simulink model "ModelLLCController"  (R2026a)
settings: Solver=ode23t  StopTime=5e-3  FixedStep=1e-4  MaxStep=1/(10*llcCompensator.resonantFrequency)  AbsTol=1e-3
PreLoadFcn:
  | % Parameterize the model
  | 
  | if ~exist('LLCDesign', 'var')
  | LLCConverterDefaultInputParameters;
  | end
undefined symbols (not defined in the file or in its folder): llcCompensator, LLCController
libraries: fl_lib x52, nesl_utility x34, ee_lib x27, ConverterLibrary x1
(part 3 of 4)

== system ModelLLCController/LLC Converter Power Circuit/LLC Primary Inverter and Resonant Tank/LLC Simplified Model/Inverter/Half Bridge Converter ==
  G1 : Inport
  G2 : Inport  Port=2
  Diode1 : fl_lib/Electrical/Electrical Elements/Diode  Vf=VfBody V  Ron=RdBody Ohm  Goff=GdBody 1/Ohm  i_specify=off  i_priority=None  i=0 A  i_nominal_specify=off  i_nominal_value=1  i_nominal_unit=A  v_specify=off  v_priority=None  v=0 V  v_nominal_specify=off  v_nominal_value=1  v_nominal_unit=V
  Diode2 : fl_lib/Electrical/Electrical Elements/Diode  Vf=VfBody V  Ron=RdBody Ohm  Goff=GdBody 1/Ohm  i_specify=off  i_priority=None  i=0 A  i_nominal_specify=off  i_nominal_value=1  i_nominal_unit=A  v_specify=off  v_priority=None  v=0 V  v_nominal_specify=off  v_nominal_value=1  v_nominal_unit=V
  Simulink-PS Converter1 : nesl_utility/Simulink-PS Converter  PhysicalDomain=network_engine_domain  SubClassName=ps_input  LeftPortType=input  RightPortType=output  PseudoPeriodic=off  Frequencies=[]  NoiseDistribution=none  NoiseParameters=[]  Unit=1  AffineConversion=off  FilteringAndDerivatives=provide  SimscapeFilterOrder=1  InputFilterTimeConstant=0.001  UdotUserProvided=0
  Simulink-PS Converter2 : nesl_utility/Simulink-PS Converter  PhysicalDomain=network_engine_domain  SubClassName=ps_input  LeftPortType=input  RightPortType=output  PseudoPeriodic=off  Frequencies=[]  NoiseDistribution=none  NoiseParameters=[]  Unit=1  AffineConversion=off  FilteringAndDerivatives=provide  SimscapeFilterOrder=1  InputFilterTimeConstant=0.001  UdotUserProvided=0
  Switch : fl_lib/Electrical/Electrical Elements/Switch  R_closed=RdsOn Ohm  G_open=GdsOff 1/Ohm  Threshold=Vth  i_specify=off  i_priority=None  i=0 A  i_nominal_specify=off  i_nominal_value=1  i_nominal_unit=A  v_specify=off  v_priority=None  v=0 V  v_nominal_specify=off  v_nominal_value=1  v_nominal_unit=V
  Switch1 : fl_lib/Electrical/Electrical Elements/Switch  R_closed=RdsOn Ohm  G_open=GdsOff 1/Ohm  Threshold=Vth  i_specify=off  i_priority=None  i=0 A  i_nominal_specify=off  i_nominal_value=1  i_nominal_unit=A  v_specify=off  v_priority=None  v=0 V  v_nominal_specify=off  v_nominal_value=1  v_nominal_unit=V
  P1 : PMIOPort  Side=Left
  N1 : PMIOPort  Port=2  Side=Left
  P2 : PMIOPort  Port=3  Side=Right
  N2 : PMIOPort  Port=4  Side=Right
  wires:
  G1/1 -> Simulink-PS Converter1/1
  G2/1 -> Simulink-PS Converter2/1
  connections:
  Switch/RConn2 -- Diode2/RConn1 -- P1/RConn1
  Diode2/LConn1 -- Switch/LConn1 -- P2/RConn1 -- Switch1/RConn2 -- Diode1/RConn1
  N1/RConn1 -- Switch1/LConn1 -- Diode1/LConn1 -- N2/RConn1
  Switch1/RConn1 -- Simulink-PS Converter2/RConn1
  Simulink-PS Converter1/RConn1 -- Switch/RConn1

== system ModelLLCController/LLC Converter Power Circuit/LLC Primary Inverter and Resonant Tank/LLC Simplified Model/Inverter/Iin ==
  Current Sensor : fl_lib/Electrical/Electrical Sensors/Current Sensor
  PS-Simulink Converter : nesl_utility/PS-Simulink Converter  PhysicalDomain=network_engine_domain  SubClassName=ps_output  LeftPortType=input  RightPortType=output  PseudoPeriodic=off  Frequencies=[]  VectorFormat=inherit  Unit=inherit  AffineConversion=off
  + : PMIOPort  Side=Left
  - : PMIOPort  Port=2  Side=Right
  I : Outport
  wires:
  PS-Simulink Converter/1 -> I/1
  connections:
  Current Sensor/RConn2 -- -/RConn1
  +/RConn1 -- Current Sensor/LConn1
  Current Sensor/RConn1 -- PS-Simulink Converter/LConn1

== system ModelLLCController/LLC Converter Power Circuit/LLC Primary Inverter and Resonant Tank/LLC Simplified Model/Inverter/Vin ==
  PS-Simulink Converter : nesl_utility/PS-Simulink Converter  PhysicalDomain=network_engine_domain  SubClassName=ps_output  LeftPortType=input  RightPortType=output  PseudoPeriodic=off  Frequencies=[]  VectorFormat=inherit  Unit=inherit  AffineConversion=off
  Voltage Sensor : fl_lib/Electrical/Electrical Sensors/Voltage Sensor
  + : PMIOPort  Side=Left
  - : PMIOPort  Port=2  Side=Right
  V : Outport
  wires:
  PS-Simulink Converter/1 -> V/1
  connections:
  Voltage Sensor/RConn2 -- -/RConn1
  Voltage Sensor/LConn1 -- +/RConn1
  PS-Simulink Converter/LConn1 -- Voltage Sensor/RConn1

== system ModelLLCController/LLC Converter Power Circuit/LLC Primary Inverter and Resonant Tank/LLC Simplified Model/Resonant Tank/Ip ==
  Current Sensor : fl_lib/Electrical/Electrical Sensors/Current Sensor
  PS-Simulink Converter : nesl_utility/PS-Simulink Converter  PhysicalDomain=network_engine_domain  SubClassName=ps_output  LeftPortType=input  RightPortType=output  PseudoPeriodic=off  Frequencies=[]  VectorFormat=inherit  Unit=inherit  AffineConversion=off
  + : PMIOPort  Side=Left
  - : PMIOPort  Port=2  Side=Right
  I : Outport
  wires:
  PS-Simulink Converter/1 -> I/1
  connections:
  Current Sensor/RConn2 -- -/RConn1
  +/RConn1 -- Current Sensor/LConn1
  Current Sensor/RConn1 -- PS-Simulink Converter/LConn1

== system ModelLLCController/LLC Converter Power Circuit/LLC Primary Inverter and Resonant Tank/LLC Simplified Model/Resonant Tank/Is ==
  Current Sensor : fl_lib/Electrical/Electrical Sensors/Current Sensor
  PS-Simulink Converter : nesl_utility/PS-Simulink Converter  PhysicalDomain=network_engine_domain  SubClassName=ps_output  LeftPortType=input  RightPortType=output  PseudoPeriodic=off  Frequencies=[]  VectorFormat=inherit  Unit=inherit  AffineConversion=off
  + : PMIOPort  Side=Left
  - : PMIOPort  Port=2  Side=Right
  I : Outport
  wires:
  PS-Simulink Converter/1 -> I/1
  connections:
  Current Sensor/RConn2 -- -/RConn1
  +/RConn1 -- Current Sensor/LConn1
  Current Sensor/RConn1 -- PS-Simulink Converter/LConn1

== system ModelLLCController/LLC Converter Power Circuit/LLC Primary Inverter and Resonant Tank/LLC Simplified Model/Resonant Tank/Vp ==
  PS-Simulink Converter : nesl_utility/PS-Simulink Converter  PhysicalDomain=network_engine_domain  SubClassName=ps_output  LeftPortType=input  RightPortType=output  PseudoPeriodic=off  Frequencies=[]  VectorFormat=inherit  Unit=inherit  AffineConversion=off
  Voltage Sensor : fl_lib/Electrical/Electrical Sensors/Voltage Sensor
  + : PMIOPort  Side=Left
  - : PMIOPort  Port=2  Side=Right
  V : Outport
  wires:
  PS-Simulink Converter/1 -> V/1
  connections:
  Voltage Sensor/RConn2 -- -/RConn1
  Voltage Sensor/LConn1 -- +/RConn1
  PS-Simulink Converter/LConn1 -- Voltage Sensor/RConn1

== system ModelLLCController/LLC Converter Power Circuit/LLC Primary Inverter and Resonant Tank/LLC Simplified Model/Resonant Tank/Vs ==
  PS-Simulink Converter : nesl_utility/PS-Simulink Converter  PhysicalDomain=network_engine_domain  SubClassName=ps_output  LeftPortType=input  RightPortType=output  PseudoPeriodic=off  Frequencies=[]  VectorFormat=inherit  Unit=inherit  AffineConversion=off
  Voltage Sensor : fl_lib/Electrical/Electrical Sensors/Voltage Sensor
  + : PMIOPort  Side=Left
  - : PMIOPort  Port=2  Side=Right
  V : Outport
  wires:
  PS-Simulink Converter/1 -> V/1
  connections:
  Voltage Sensor/RConn2 -- -/RConn1
  Voltage Sensor/LConn1 -- +/RConn1
  PS-Simulink Converter/LConn1 -- Voltage Sensor/RConn1

== system ModelLLCController/LLC Converter Power Circuit/Rectifier/Rectifier Bridge/Centre-Tap Ideal Diode/Is ==
  Current Sensor : fl_lib/Electrical/Electrical Sensors/Current Sensor
  PS-Simulink Converter : nesl_utility/PS-Simulink Converter  PhysicalDomain=network_engine_domain  SubClassName=ps_output  LeftPortType=input  RightPortType=output  PseudoPeriodic=off  Frequencies=[]  VectorFormat=inherit  Unit=inherit  AffineConversion=off
  + : PMIOPort  Side=Left
  - : PMIOPort  Port=2  Side=Right
  I : Outport
  wires:
  PS-Simulink Converter/1 -> I/1
  connections:
  Current Sensor/RConn2 -- -/RConn1
  +/RConn1 -- Current Sensor/LConn1
  Current Sensor/RConn1 -- PS-Simulink Converter/LConn1

== system ModelLLCController/LLC Converter Power Circuit/Rectifier/Rectifier Bridge/Centre-Tap Tabulated Diode/Is ==
  Current Sensor : fl_lib/Electrical/Electrical Sensors/Current Sensor
  PS-Simulink Converter : nesl_utility/PS-Simulink Converter  PhysicalDomain=network_engine_domain  SubClassName=ps_output  LeftPortType=input  RightPortType=output  PseudoPeriodic=off  Frequencies=[]  VectorFormat=inherit  Unit=inherit  AffineConversion=off
  + : PMIOPort  Side=Left
  - : PMIOPort  Port=2  Side=Right
  I : Outport
  wires:
  PS-Simulink Converter/1 -> I/1
  connections:
  Current Sensor/RConn2 -- -/RConn1
  +/RConn1 -- Current Sensor/LConn1
  Current Sensor/RConn1 -- PS-Simulink Converter/LConn1

== system ModelLLCController/LLC Converter Power Circuit/Rectifier/Rectifier Bridge/Full Bridge Ideal Diode/Is ==
  Current Sensor : fl_lib/Electrical/Electrical Sensors/Current Sensor
  PS-Simulink Converter : nesl_utility/PS-Simulink Converter  PhysicalDomain=network_engine_domain  SubClassName=ps_output  LeftPortType=input  RightPortType=output  PseudoPeriodic=off  Frequencies=[]  VectorFormat=inherit  Unit=inherit  AffineConversion=off
  + : PMIOPort  Side=Left
  - : PMIOPort  Port=2  Side=Right
  I : Outport
  wires:
  PS-Simulink Converter/1 -> I/1
  connections:
  Current Sensor/RConn2 -- -/RConn1
  +/RConn1 -- Current Sensor/LConn1
  Current Sensor/RConn1 -- PS-Simulink Converter/LConn1

== system ModelLLCController/LLC Converter Power Circuit/Rectifier/Rectifier Bridge/Full Bridge Tabulated Diode/Is ==
  Current Sensor : fl_lib/Electrical/Electrical Sensors/Current Sensor
  PS-Simulink Converter : nesl_utility/PS-Simulink Converter  PhysicalDomain=network_engine_domain  SubClassName=ps_output  LeftPortType=input  RightPortType=output  PseudoPeriodic=off  Frequencies=[]  VectorFormat=inherit  Unit=inherit  AffineConversion=off
  + : PMIOPort  Side=Left
  - : PMIOPort  Port=2  Side=Right
  I : Outport
  wires:
  PS-Simulink Converter/1 -> I/1
  connections:
  Current Sensor/RConn2 -- -/RConn1
  +/RConn1 -- Current Sensor/LConn1
  Current Sensor/RConn1 -- PS-Simulink Converter/LConn1

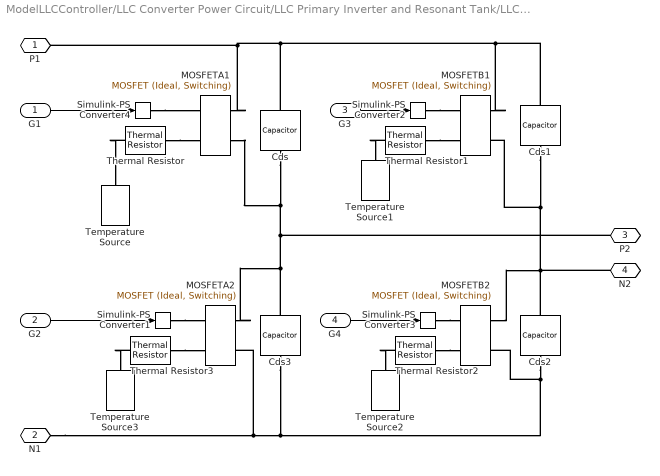
== system ModelLLCController/LLC Converter Power Circuit/LLC Primary Inverter and Resonant Tank/LLC Detailed Model/Inverter/Primary Inverter/Full Bridge with Thermal ==
  G1 : Inport
  G2 : Inport  Port=2
  G3 : Inport  Port=3
  G4 : Inport  Port=4
  Cds{,1..3} (4 alike) : fl_lib/Electrical/Electrical Elements/Capacitor  c=Cdsparasitic F  r=0.05 Ohm  g=1e-5 1/Ohm  i_specify=off  i_priority=None  i=0 A  i_nominal_specify=off  i_nominal_value=1  i_nominal_unit=A  v_specify=off  v_priority=None  v=0 V  v_nominal_specify=off  v_nominal_value=1  v_nominal_unit=V  vc_specify=off  vc_priority=High  vc=0 V  vc_nominal_specify=off  vc_nominal_value=1  vc_nominal_unit=V
  MOSFETA1 : ee_lib/Semiconductors & Converters/MOSFET (Ideal, Switching)  PartSpecification="{\"CollectionId\":\"SimscapeElectrical\",\"CollectionVersion\":\"1.0.0\",\"DatasetId\":\"STMicroelectronics|SCTH35N65G2V-7|simscape.electrical.mosfetIdealSwitching\",\"DisplayName\":\"STMicroelectronics:SCTH35N65G2V-7\"}"  port_option=ee.enum.controlport.ps  Rds=0.08 % Datasheet derived Ohm  Goff=1e-08 % Datasheet derived 1/Ohm  Vth=3.2 % Datasheet derived V  diode_param=ee.enum.semiconductors.protectionDiode.nodynamics  diode_Vf=2.72 % Datasheet derived V  diode_Ron=0.025 % Datasheet derived Ohm  diode_Goff=1e-05 % Library default 1/Ohm  diode_C=50e-9 % Parameter not set F  diode_iRM=-235 % Parameter not set A  diode_iF=300 % Parameter not set A  diode_idot=-50 % Parameter not set A/us  diode_trr_param=ee.enum.converters.diodeReverseParam.trr_factor  diode_trr_factor=3 % Parameter not set  diode_trr=15 % Parameter not set us  diode_Qrr=1500 % Parameter not set s*uA  ids_specify=off  ids_priority=None  ids=0 A  ids_nominal_specify=off  ids_nominal_value=1  ids_nominal_unit=A  vds_specify=off  vds_priority=None  vds=0 V  vds_nominal_specify=off  vds_nominal_value=1  vds_nominal_unit=V  vgs_specify=off  vgs_priority=None  vgs=0 V  vgs_nominal_specify=off  vgs_nominal_value=1  vgs_nominal_unit=V  thermal_loss_option=ee.enum.converters.thermalLossOption.tabulated2d  Von_data=[0 0.25 0.49 0.74 1.02 1.3 1.58 1.89 2.2 2.49 2.76 3.03 3.33 3.65 3.98 4.34 4.71 5.08 5.47 5.86 6.27 6.68 7.18 7.79;0 0.33 0.66 0.98 1.34 1.71 2.08 2.47 2.92 3.36 3.82 4.33 4.85 5.38 6.06 6.73 7.54 8.48 9.52 10.82 12.49 14.66 16.83 18.99] % Datasheet derived V  Tj=[25 175] % Datasheet derived degC  Iout_data=[0 4.34 8.68 13.02 17.36 21.69 26.03 30.37 34.71 39.05 43.39 47.73 52.07 56.41 60.74 65.08 69.42 73.76 78.1 82.44 86.78 91.12 95.46 99.79] % Datasheet derived A  tabulateWithVds=false % Parameter not set  Eon_data=[48.85 51.27 53.69 56.12 58.54 60.96 63.38 65.81 68.23 70.65 73.07 75.5 77.92 80.34 82.76 85.19 87.61 90.03 92.45 96.36 101.18 106.01 110.83 115.66 120.48 125.3 130.13 134.95 139.78 144.6 149.42 154.25 160.12 167.74 175.35 182.96 190.58 198.19 205.81 213.42 221.04 228.65 236.26 243.88 251.49 259.11 266.72 278.95 292.18 305.42 318.66 331.89 345.13 358.37 371.61 384.84 398.08 411.32 424.56 439.44 457.69 475.94 494.19 512.43 530.68 548.93 568.13 588.61 609.09 629.57 650.05 670.53] % Datasheet derived uJ  Eoff_data=[31.1 31.28 31.47 31.66 31.84 32.03 32.21 32.4 32.58 32.77 32.96 33.14 33.33 33.51 33.7 33.89 34.07 37.14 40.34 43.53 46.72 49.91 53.1 56.29 59.48 62.68 65.87 69.67 75.6 81.53 87.46 93.39 99.32 105.25 111.18 117.11 123.04 128.97 134.9 141.66 148.96 156.26 163.56 170.86 178.16 185.46 192.76 200.06 207.36 214.66 222.22 231.42 240.63 249.83 259.04 268.24 277.45 286.65 295.86 305.06 314.27 323.6 332.99 342.39 351.78 361.17 370.56 379.95 389.35 398.74 408.13 417.52] % Datasheet derived uJ  Eon_data_3D=[zeros(2, 5, 3)] % Parameter not set J  Eoff_data_3D=[zeros(2, 5, 3)] % Parameter not set J  Tj_loss=25 % Datasheet derived degC  Iout_data_loss=[0 1.12 2.24 3.36 4.47 5.59 6.71 7.83 8.95 10.07 11.18 12.3 13.42 14.54 15.66 16.78 17.9 19.01 20.13 21.25 22.37 23.49 24.61 25.72 26.84 27.96 29.08 30.2 31.32 32.44 33.55 34.67 35.79 36.91 38.03 39.15 40.26 41.38 42.5 43.62 44.74 45.86 46.97 48.09 49.21 50.33 51.45 52.57 53.69 54.8 55.92 57.04 58.16 59.28 60.4 61.51 62.63 63.75 64.87 65.99 67.11 68.23 69.34 70.46 71.58 72.7 73.82 74.94 76.05 77.17 78.29 79.41] % Datasheet derived A  Vds_loss=[0, 150, 300] % Parameter not set V  Eon_scalar=22.86e-3 % Parameter not set J  Eoff_scalar=17.14e-3 % Parameter not set J  Voff=400 % Datasheet derived V  Iout_scalar=600 % Parameter not set A  useCurrentFromPreviousCycle=false % Parameter not set  useVoltageFromPreviousCycle=false % Parameter not set  diodeModelType=ee.enum.converters.diodeModelType.tabulated  diodeTableType=ee.enum.diode.tableType.IfMat  diode_ReverseIVType=ee.enum.diode.diodeReverseIV.constant  diode_IfMat=[0 0.1665 0.2493 2.6035 11.0361 27.1534 51.6742 89.05;0 0.3874 0.8255 4.4328 17.0798 39.5683 67.6172 103.3819] % Datasheet derived A  diode_VfMat=[.9, 1.15, 1.25, 1.5, 1.75, 2.17, 2.6, 2.85; .58, .68, .75, 1.1, 1.38, 1.77, 2.27, 2.7] % Parameter not set V  diode_TjVec=[25 175] % Datasheet derived degC  diode_VfVec=[0 1 1.99 2.99 3.98 4.98 5.97 6.97] % Datasheet derived V  diode_IfVec=[.1, .2, .5, 1, 2, 4, 7, 10] % Parameter not set A  diode_IrMat=[1e-06, 2e-06, 5e-06, 1e-05, 2.5e-05, 5e-05, .0001; 2e-06, 5e-06, 1e-05, 4e-05, 8e-05, .0002, .0005] % Parameter not set A  diode_VrMat=[10, 100, 200, 250, 300, 325, 350; 10, 70, 160, 220, 270, 300, 320] % Parameter not set V  diode_VrVec=[10, 20, 40, 50, 70, 80, 100] % Parameter not set V  diode_IrVec=[1e-06, 2e-06, 5e-06, 1e-05, 2e-05, 5e-05, .0001] % Parameter not set A  diode_Vr=-600 % Parameter not set V  diode_Ls=150 % Parameter not set nH  diode_Erec=0.03 % Parameter not set J  diode_rec_loss_model=ee.enum.diode.reverseRecoveryModel.fixed  diode_ErecVal=0 % Parameter not set J  diode_scaleWithIandV=false  diode_ErecMat=zeros(2, 3) % Parameter not set J  diodeErecMat3D=zeros(2, 3, 2) J  diode_TjrecVec=[298.15, 398.15] % Parameter not set K  diode_IfrecVec=[.1, 1, 10] % Parameter not set A  diodeVrecVec=[0, 100] V  diode_IrecVal=10 % Parameter not set A  diode_VrecVal=10 % Parameter not set V  diode_tFilter=1 / 1000 / 100 % Parameter not set s  separateThermalPortForDiode=false % Parameter not set  thermal_network_parameterization=ee.enum.thermalNetworkTopology.external  Rth=[.03, .2] % Parameter not set K/W  Rth_Cauer=[.03, .1, .2] % Parameter not set K/W  Rth_Foster=[.08, .14, .22, .16] % Parameter not set K/W  thermal_mass_parameterization=ee.enum.thermalNetwork.timeconstant  thermal_mass=[3, 25] % Parameter not set J/K  thermal_mass_Cauer=[3, 10, 25] % Parameter not set J/K  thermal_mass_Foster=[.001, .005, .05, .5] % Parameter not set J/K  thermal_time_constant=[.1, 5] % Parameter not set s  thermal_time_constant_Cauer=[.1, 1, 5] % Parameter not set s  thermal_time_constant_Foster=[7e-05, .0007, .01, .08] % Parameter not set s  thermal_mass_initial_temperatures=[25, 25] % Parameter not set degC  thermal_mass_initial_temperatures_Cauer=[25, 25, 25] % Parameter not set degC  junction_thermal_mass=1.29 % Datasheet derived J/K  Tvec_initial_Foster=[25, 25, 25, 25] % Parameter not set degC  RthDiode=[.03, .2] % Parameter not set K/W  RthCauerDiode=[.03, .1, .2] % Parameter not set K/W  RthFosterDiode=[.03, .2] % Parameter not set K/W  thermalMassDiode=[3, 25] % Parameter not set J/K  thermalMassCauerDiode=[3, 10, 25] % Parameter not set J/K  thermalMassFosterDiode=[33, 50] % Parameter not set J/K  thermalTauDiode=[.1, 5] % Parameter not set s  thermalTauCauerDiode=[.1, 1, 5] % Parameter not set s  thermalTauFosterDiode=[1, 10] % Parameter not set s  thermalMassInitTempDiode=[25, 25] % Parameter not set degC  thermalMassInitTempCauerDiode=[25, 25, 25] % Parameter not set degC  junctionthermalMassDiode=0.1 % Parameter not set J/K  TVecInitialFosterDiode=[25, 25, 25, 25] % Parameter not set degC  no_thermal_network=0 % Parameter not set  mosfet_junction_temperature_specify=on  mosfet_junction_temperature_priority=High  mosfet_junction_temperature=simTempPri_K K  mosfet_junction_temperature_nominal_specify=off  mosfet_junction_temperature_nominal_value=1  mosfet_junction_temperature_nominal_unit=degC  diode_junction_temperature_specify=off  diode_junction_temperature_priority=None  diode_junction_temperature=simTempPri_K K  diode_junction_temperature_nominal_specify=off  diode_junction_temperature_nominal_value=1  diode_junction_temperature_nominal_unit=degC  Qj_specify=off  Qj_priority=None  Qj=0 W  Qj_nominal_specify=off  Qj_nominal_value=1  Qj_nominal_unit=W  accumulatedSwitchingLosses_specify=off  accumulatedSwitchingLosses_priority=None  accumulatedSwitchingLosses=0 J
      settings: AttributesFormatString=STMicroelectronics:SCTH35N65G2V-7
  MOSFETA2 : ee_lib/Semiconductors & Converters/MOSFET (Ideal, Switching)  PartSpecification="{\"DatasetId\":\"STMicroelectronics|SCTH35N65G2V-7|simscape.electrical.mosfetIdealSwitching\",\"DisplayName\":\"STMicroelectronics:SCTH35N65G2V-7\"}"  port_option=ee.enum.controlport.ps  Rds=0.08 % Datasheet derived Ohm  Goff=1e-08 % Datasheet derived 1/Ohm  Vth=3.2 % Datasheet derived V  diode_param=ee.enum.semiconductors.protectionDiode.nodynamics  diode_Vf=2.72 % Datasheet derived V  diode_Ron=0.025 % Datasheet derived Ohm  diode_Goff=1e-05 % Library default 1/Ohm  diode_C=50e-9 % Parameter not set F  diode_iRM=-235 % Parameter not set A  diode_iF=300 % Parameter not set A  diode_idot=-50 % Parameter not set A/us  diode_trr_param=ee.enum.converters.diodeReverseParam.trr_factor  diode_trr_factor=3 % Parameter not set  diode_trr=15 % Parameter not set us  diode_Qrr=1500 % Parameter not set s*uA  ids_specify=off  ids_priority=None  ids=0 A  ids_nominal_specify=off  ids_nominal_value=1  ids_nominal_unit=A  vds_specify=off  vds_priority=None  vds=0 V  vds_nominal_specify=off  vds_nominal_value=1  vds_nominal_unit=V  vgs_specify=off  vgs_priority=None  vgs=0 V  vgs_nominal_specify=off  vgs_nominal_value=1  vgs_nominal_unit=V  thermal_loss_option=ee.enum.converters.thermalLossOption.tabulated2d  Von_data=[0 0.25 0.49 0.74 1.02 1.3 1.58 1.89 2.2 2.49 2.76 3.03 3.33 3.65 3.98 4.34 4.71 5.08 5.47 5.86 6.27 6.68 7.18 7.79;0 0.33 0.66 0.98 1.34 1.71 2.08 2.47 2.92 3.36 3.82 4.33 4.85 5.38 6.06 6.73 7.54 8.48 9.52 10.82 12.49 14.66 16.83 18.99] % Datasheet derived V  Tj=[25 175] % Datasheet derived degC  Iout_data=[0 4.34 8.68 13.02 17.36 21.69 26.03 30.37 34.71 39.05 43.39 47.73 52.07 56.41 60.74 65.08 69.42 73.76 78.1 82.44 86.78 91.12 95.46 99.79] % Datasheet derived A  tabulateWithVds=false % Parameter not set  Eon_data=[48.85 51.27 53.69 56.12 58.54 60.96 63.38 65.81 68.23 70.65 73.07 75.5 77.92 80.34 82.76 85.19 87.61 90.03 92.45 96.36 101.18 106.01 110.83 115.66 120.48 125.3 130.13 134.95 139.78 144.6 149.42 154.25 160.12 167.74 175.35 182.96 190.58 198.19 205.81 213.42 221.04 228.65 236.26 243.88 251.49 259.11 266.72 278.95 292.18 305.42 318.66 331.89 345.13 358.37 371.61 384.84 398.08 411.32 424.56 439.44 457.69 475.94 494.19 512.43 530.68 548.93 568.13 588.61 609.09 629.57 650.05 670.53] % Datasheet derived uJ  Eoff_data=[31.1 31.28 31.47 31.66 31.84 32.03 32.21 32.4 32.58 32.77 32.96 33.14 33.33 33.51 33.7 33.89 34.07 37.14 40.34 43.53 46.72 49.91 53.1 56.29 59.48 62.68 65.87 69.67 75.6 81.53 87.46 93.39 99.32 105.25 111.18 117.11 123.04 128.97 134.9 141.66 148.96 156.26 163.56 170.86 178.16 185.46 192.76 200.06 207.36 214.66 222.22 231.42 240.63 249.83 259.04 268.24 277.45 286.65 295.86 305.06 314.27 323.6 332.99 342.39 351.78 361.17 370.56 379.95 389.35 398.74 408.13 417.52] % Datasheet derived uJ  Eon_data_3D=[zeros(2, 5, 3)] % Parameter not set J  Eoff_data_3D=[zeros(2, 5, 3)] % Parameter not set J  Tj_loss=25 % Datasheet derived degC  Iout_data_loss=[0 1.12 2.24 3.36 4.47 5.59 6.71 7.83 8.95 10.07 11.18 12.3 13.42 14.54 15.66 16.78 17.9 19.01 20.13 21.25 22.37 23.49 24.61 25.72 26.84 27.96 29.08 30.2 31.32 32.44 33.55 34.67 35.79 36.91 38.03 39.15 40.26 41.38 42.5 43.62 44.74 45.86 46.97 48.09 49.21 50.33 51.45 52.57 53.69 54.8 55.92 57.04 58.16 59.28 60.4 61.51 62.63 63.75 64.87 65.99 67.11 68.23 69.34 70.46 71.58 72.7 73.82 74.94 76.05 77.17 78.29 79.41] % Datasheet derived A  Vds_loss=[0, 150, 300] % Parameter not set V  Eon_scalar=22.86e-3 % Parameter not set J  Eoff_scalar=17.14e-3 % Parameter not set J  Voff=400 % Datasheet derived V  Iout_scalar=600 % Parameter not set A  useCurrentFromPreviousCycle=false % Parameter not set  useVoltageFromPreviousCycle=false % Parameter not set  diodeModelType=ee.enum.converters.diodeModelType.tabulated  diodeTableType=ee.enum.diode.tableType.IfMat  diode_ReverseIVType=ee.enum.diode.diodeReverseIV.constant  diode_IfMat=[0 0.1665 0.2493 2.6035 11.0361 27.1534 51.6742 89.05;0 0.3874 0.8255 4.4328 17.0798 39.5683 67.6172 103.3819] % Datasheet derived A  diode_VfMat=[.9, 1.15, 1.25, 1.5, 1.75, 2.17, 2.6, 2.85; .58, .68, .75, 1.1, 1.38, 1.77, 2.27, 2.7] % Parameter not set V  diode_TjVec=[25 175] % Datasheet derived degC  diode_VfVec=[0 1 1.99 2.99 3.98 4.98 5.97 6.97] % Datasheet derived V  diode_IfVec=[.1, .2, .5, 1, 2, 4, 7, 10] % Parameter not set A  diode_IrMat=[1e-06, 2e-06, 5e-06, 1e-05, 2.5e-05, 5e-05, .0001; 2e-06, 5e-06, 1e-05, 4e-05, 8e-05, .0002, .0005] % Parameter not set A  diode_VrMat=[10, 100, 200, 250, 300, 325, 350; 10, 70, 160, 220, 270, 300, 320] % Parameter not set V  diode_VrVec=[10, 20, 40, 50, 70, 80, 100] % Parameter not set V  diode_IrVec=[1e-06, 2e-06, 5e-06, 1e-05, 2e-05, 5e-05, .0001] % Parameter not set A  diode_Vr=-600 % Parameter not set V  diode_Ls=150 % Parameter not set nH  diode_Erec=0.03 % Parameter not set J  diode_rec_loss_model=ee.enum.diode.reverseRecoveryModel.fixed  diode_ErecVal=0 % Parameter not set J  diode_scaleWithIandV=false  diode_ErecMat=zeros(2, 3) % Parameter not set J  diodeErecMat3D=zeros(2, 3, 2) J  diode_TjrecVec=[298.15, 398.15] % Parameter not set K  diode_IfrecVec=[.1, 1, 10] % Parameter not set A  diodeVrecVec=[0, 100] V  diode_IrecVal=10 % Parameter not set A  diode_VrecVal=10 % Parameter not set V  diode_tFilter=1 / 1000 / 100 % Parameter not set s  separateThermalPortForDiode=false % Parameter not set  thermal_network_parameterization=ee.enum.thermalNetworkTopology.external  Rth=[.03, .2] % Parameter not set K/W  Rth_Cauer=[.03, .1, .2] % Parameter not set K/W  Rth_Foster=[.08, .14, .22, .16] % Parameter not set K/W  thermal_mass_parameterization=ee.enum.thermalNetwork.timeconstant  thermal_mass=[3, 25] % Parameter not set J/K  thermal_mass_Cauer=[3, 10, 25] % Parameter not set J/K  thermal_mass_Foster=[.001, .005, .05, .5] % Parameter not set J/K  thermal_time_constant=[.1, 5] % Parameter not set s  thermal_time_constant_Cauer=[.1, 1, 5] % Parameter not set s  thermal_time_constant_Foster=[7e-05, .0007, .01, .08] % Parameter not set s  thermal_mass_initial_temperatures=[25, 25] % Parameter not set degC  thermal_mass_initial_temperatures_Cauer=[25, 25, 25] % Parameter not set degC  junction_thermal_mass=1.29 % Datasheet derived J/K  Tvec_initial_Foster=[25, 25, 25, 25] % Parameter not set degC  RthDiode=[.03, .2] % Parameter not set K/W  RthCauerDiode=[.03, .1, .2] % Parameter not set K/W  RthFosterDiode=[.03, .2] % Parameter not set K/W  thermalMassDiode=[3, 25] % Parameter not set J/K  thermalMassCauerDiode=[3, 10, 25] % Parameter not set J/K  thermalMassFosterDiode=[33, 50] % Parameter not set J/K  thermalTauDiode=[.1, 5] % Parameter not set s  thermalTauCauerDiode=[.1, 1, 5] % Parameter not set s  thermalTauFosterDiode=[1, 10] % Parameter not set s  thermalMassInitTempDiode=[25, 25] % Parameter not set degC  thermalMassInitTempCauerDiode=[25, 25, 25] % Parameter not set degC  junctionthermalMassDiode=0.1 % Parameter not set J/K  TVecInitialFosterDiode=[25, 25, 25, 25] % Parameter not set degC  no_thermal_network=0 % Parameter not set  mosfet_junction_temperature_specify=on  mosfet_junction_temperature_priority=High  mosfet_junction_temperature=simTempPri_K K  mosfet_junction_temperature_nominal_specify=off  mosfet_junction_temperature_nominal_value=1  mosfet_junction_temperature_nominal_unit=degC  diode_junction_temperature_specify=off  diode_junction_temperature_priority=None  diode_junction_temperature=simTempPri_K K  diode_junction_temperature_nominal_specify=off  diode_junction_temperature_nominal_value=1  diode_junction_temperature_nominal_unit=degC  Qj_specify=off  Qj_priority=None  Qj=0 W  Qj_nominal_specify=off  Qj_nominal_value=1  Qj_nominal_unit=W  accumulatedSwitchingLosses_specify=off  accumulatedSwitchingLosses_priority=None  accumulatedSwitchingLosses=0 J
      settings: AttributesFormatString=STMicroelectronics:SCTH35N65G2V-7
  MOSFETB1 : ee_lib/Semiconductors & Converters/MOSFET (Ideal, Switching)  PartSpecification="{\"CollectionId\":\"SimscapeElectrical\",\"DatasetId\":\"STMicroelectronics|SCTH35N65G2V-7|simscape.electrical.mosfetIdealSwitching\",\"DisplayName\":\"STMicroelectronics:SCTH35N65G2V-7\"}"  port_option=ee.enum.controlport.ps  Rds=0.08 % Datasheet derived Ohm  Goff=1e-08 % Datasheet derived 1/Ohm  Vth=3.2 % Datasheet derived V  diode_param=ee.enum.semiconductors.protectionDiode.nodynamics  diode_Vf=2.72 % Datasheet derived V  diode_Ron=0.025 % Datasheet derived Ohm  diode_Goff=1e-05 % Library default 1/Ohm  diode_C=50e-9 % Parameter not set F  diode_iRM=-235 % Parameter not set A  diode_iF=300 % Parameter not set A  diode_idot=-50 % Parameter not set A/us  diode_trr_param=ee.enum.converters.diodeReverseParam.trr_factor  diode_trr_factor=3 % Parameter not set  diode_trr=15 % Parameter not set us  diode_Qrr=1500 % Parameter not set s*uA  ids_specify=off  ids_priority=None  ids=0 A  ids_nominal_specify=off  ids_nominal_value=1  ids_nominal_unit=A  vds_specify=off  vds_priority=None  vds=0 V  vds_nominal_specify=off  vds_nominal_value=1  vds_nominal_unit=V  vgs_specify=off  vgs_priority=None  vgs=0 V  vgs_nominal_specify=off  vgs_nominal_value=1  vgs_nominal_unit=V  thermal_loss_option=ee.enum.converters.thermalLossOption.tabulated2d  Von_data=[0 0.25 0.49 0.74 1.02 1.3 1.58 1.89 2.2 2.49 2.76 3.03 3.33 3.65 3.98 4.34 4.71 5.08 5.47 5.86 6.27 6.68 7.18 7.79;0 0.33 0.66 0.98 1.34 1.71 2.08 2.47 2.92 3.36 3.82 4.33 4.85 5.38 6.06 6.73 7.54 8.48 9.52 10.82 12.49 14.66 16.83 18.99] % Datasheet derived V  Tj=[25 175] % Datasheet derived degC  Iout_data=[0 4.34 8.68 13.02 17.36 21.69 26.03 30.37 34.71 39.05 43.39 47.73 52.07 56.41 60.74 65.08 69.42 73.76 78.1 82.44 86.78 91.12 95.46 99.79] % Datasheet derived A  tabulateWithVds=false % Parameter not set  Eon_data=[48.85 51.27 53.69 56.12 58.54 60.96 63.38 65.81 68.23 70.65 73.07 75.5 77.92 80.34 82.76 85.19 87.61 90.03 92.45 96.36 101.18 106.01 110.83 115.66 120.48 125.3 130.13 134.95 139.78 144.6 149.42 154.25 160.12 167.74 175.35 182.96 190.58 198.19 205.81 213.42 221.04 228.65 236.26 243.88 251.49 259.11 266.72 278.95 292.18 305.42 318.66 331.89 345.13 358.37 371.61 384.84 398.08 411.32 424.56 439.44 457.69 475.94 494.19 512.43 530.68 548.93 568.13 588.61 609.09 629.57 650.05 670.53] % Datasheet derived uJ  Eoff_data=[31.1 31.28 31.47 31.66 31.84 32.03 32.21 32.4 32.58 32.77 32.96 33.14 33.33 33.51 33.7 33.89 34.07 37.14 40.34 43.53 46.72 49.91 53.1 56.29 59.48 62.68 65.87 69.67 75.6 81.53 87.46 93.39 99.32 105.25 111.18 117.11 123.04 128.97 134.9 141.66 148.96 156.26 163.56 170.86 178.16 185.46 192.76 200.06 207.36 214.66 222.22 231.42 240.63 249.83 259.04 268.24 277.45 286.65 295.86 305.06 314.27 323.6 332.99 342.39 351.78 361.17 370.56 379.95 389.35 398.74 408.13 417.52] % Datasheet derived uJ  Eon_data_3D=[zeros(2, 5, 3)] % Parameter not set J  Eoff_data_3D=[zeros(2, 5, 3)] % Parameter not set J  Tj_loss=25 % Datasheet derived degC  Iout_data_loss=[0 1.12 2.24 3.36 4.47 5.59 6.71 7.83 8.95 10.07 11.18 12.3 13.42 14.54 15.66 16.78 17.9 19.01 20.13 21.25 22.37 23.49 24.61 25.72 26.84 27.96 29.08 30.2 31.32 32.44 33.55 34.67 35.79 36.91 38.03 39.15 40.26 41.38 42.5 43.62 44.74 45.86 46.97 48.09 49.21 50.33 51.45 52.57 53.69 54.8 55.92 57.04 58.16 59.28 60.4 61.51 62.63 63.75 64.87 65.99 67.11 68.23 69.34 70.46 71.58 72.7 73.82 74.94 76.05 77.17 78.29 79.41] % Datasheet derived A  Vds_loss=[0, 150, 300] % Parameter not set V  Eon_scalar=22.86e-3 % Parameter not set J  Eoff_scalar=17.14e-3 % Parameter not set J  Voff=400 % Datasheet derived V  Iout_scalar=600 % Parameter not set A  useCurrentFromPreviousCycle=false % Parameter not set  useVoltageFromPreviousCycle=false % Parameter not set  diodeModelType=ee.enum.converters.diodeModelType.tabulated  diodeTableType=ee.enum.diode.tableType.IfMat  diode_ReverseIVType=ee.enum.diode.diodeReverseIV.constant  diode_IfMat=[0 0.1665 0.2493 2.6035 11.0361 27.1534 51.6742 89.05;0 0.3874 0.8255 4.4328 17.0798 39.5683 67.6172 103.3819] % Datasheet derived A  diode_VfMat=[.9, 1.15, 1.25, 1.5, 1.75, 2.17, 2.6, 2.85; .58, .68, .75, 1.1, 1.38, 1.77, 2.27, 2.7] % Parameter not set V  diode_TjVec=[25 175] % Datasheet derived degC  diode_VfVec=[0 1 1.99 2.99 3.98 4.98 5.97 6.97] % Datasheet derived V  diode_IfVec=[.1, .2, .5, 1, 2, 4, 7, 10] % Parameter not set A  diode_IrMat=[1e-06, 2e-06, 5e-06, 1e-05, 2.5e-05, 5e-05, .0001; 2e-06, 5e-06, 1e-05, 4e-05, 8e-05, .0002, .0005] % Parameter not set A  diode_VrMat=[10, 100, 200, 250, 300, 325, 350; 10, 70, 160, 220, 270, 300, 320] % Parameter not set V  diode_VrVec=[10, 20, 40, 50, 70, 80, 100] % Parameter not set V  diode_IrVec=[1e-06, 2e-06, 5e-06, 1e-05, 2e-05, 5e-05, .0001] % Parameter not set A  diode_Vr=-600 % Parameter not set V  diode_Ls=150 % Parameter not set nH  diode_Erec=0.03 % Parameter not set J  diode_rec_loss_model=ee.enum.diode.reverseRecoveryModel.fixed  diode_ErecVal=0 % Parameter not set J  diode_scaleWithIandV=false  diode_ErecMat=zeros(2, 3) % Parameter not set J  diodeErecMat3D=zeros(2, 3, 2) J  diode_TjrecVec=[298.15, 398.15] % Parameter not set K  diode_IfrecVec=[.1, 1, 10] % Parameter not set A  diodeVrecVec=[0, 100] V  diode_IrecVal=10 % Parameter not set A  diode_VrecVal=10 % Parameter not set V  diode_tFilter=1 / 1000 / 100 % Parameter not set s  separateThermalPortForDiode=false % Parameter not set  thermal_network_parameterization=ee.enum.thermalNetworkTopology.external  Rth=[.03, .2] % Parameter not set K/W  Rth_Cauer=[.03, .1, .2] % Parameter not set K/W  Rth_Foster=[.08, .14, .22, .16] % Parameter not set K/W  thermal_mass_parameterization=ee.enum.thermalNetwork.timeconstant  thermal_mass=[3, 25] % Parameter not set J/K  thermal_mass_Cauer=[3, 10, 25] % Parameter not set J/K  thermal_mass_Foster=[.001, .005, .05, .5] % Parameter not set J/K  thermal_time_constant=[.1, 5] % Parameter not set s  thermal_time_constant_Cauer=[.1, 1, 5] % Parameter not set s  thermal_time_constant_Foster=[7e-05, .0007, .01, .08] % Parameter not set s  thermal_mass_initial_temperatures=[25, 25] % Parameter not set degC  thermal_mass_initial_temperatures_Cauer=[25, 25, 25] % Parameter not set degC  junction_thermal_mass=1.29 % Datasheet derived J/K  Tvec_initial_Foster=[25, 25, 25, 25] % Parameter not set degC  RthDiode=[.03, .2] % Parameter not set K/W  RthCauerDiode=[.03, .1, .2] % Parameter not set K/W  RthFosterDiode=[.03, .2] % Parameter not set K/W  thermalMassDiode=[3, 25] % Parameter not set J/K  thermalMassCauerDiode=[3, 10, 25] % Parameter not set J/K  thermalMassFosterDiode=[33, 50] % Parameter not set J/K  thermalTauDiode=[.1, 5] % Parameter not set s  thermalTauCauerDiode=[.1, 1, 5] % Parameter not set s  thermalTauFosterDiode=[1, 10] % Parameter not set s  thermalMassInitTempDiode=[25, 25] % Parameter not set degC  thermalMassInitTempCauerDiode=[25, 25, 25] % Parameter not set degC  junctionthermalMassDiode=0.1 % Parameter not set J/K  TVecInitialFosterDiode=[25, 25, 25, 25] % Parameter not set degC  no_thermal_network=0 % Parameter not set  mosfet_junction_temperature_specify=on  mosfet_junction_temperature_priority=High  mosfet_junction_temperature=simTempPri_K K  mosfet_junction_temperature_nominal_specify=off  mosfet_junction_temperature_nominal_value=1  mosfet_junction_temperature_nominal_unit=degC  diode_junction_temperature_specify=off  diode_junction_temperature_priority=None  diode_junction_temperature=simTempPri_K K  diode_junction_temperature_nominal_specify=off  diode_junction_temperature_nominal_value=1  diode_junction_temperature_nominal_unit=degC  Qj_specify=off  Qj_priority=None  Qj=0 W  Qj_nominal_specify=off  Qj_nominal_value=1  Qj_nominal_unit=W  accumulatedSwitchingLosses_specify=off  accumulatedSwitchingLosses_priority=None  accumulatedSwitchingLosses=0 J
      settings: AttributesFormatString=STMicroelectronics:SCTH35N65G2V-7
  MOSFETB2 : ee_lib/Semiconductors & Converters/MOSFET (Ideal, Switching)  PartSpecification="{\"DatasetId\":\"STMicroelectronics|SCTH35N65G2V-7|simscape.electrical.mosfetIdealSwitching\",\"DisplayName\":\"STMicroelectronics:SCTH35N65G2V-7\"}"  port_option=ee.enum.controlport.ps  Rds=0.08 % Datasheet derived Ohm  Goff=1e-08 % Datasheet derived 1/Ohm  Vth=3.2 % Datasheet derived V  diode_param=ee.enum.semiconductors.protectionDiode.nodynamics  diode_Vf=2.72 % Datasheet derived V  diode_Ron=0.025 % Datasheet derived Ohm  diode_Goff=1e-05 % Library default 1/Ohm  diode_C=50e-9 % Parameter not set F  diode_iRM=-235 % Parameter not set A  diode_iF=300 % Parameter not set A  diode_idot=-50 % Parameter not set A/us  diode_trr_param=ee.enum.converters.diodeReverseParam.trr_factor  diode_trr_factor=3 % Parameter not set  diode_trr=15 % Parameter not set us  diode_Qrr=1500 % Parameter not set s*uA  ids_specify=off  ids_priority=None  ids=0 A  ids_nominal_specify=off  ids_nominal_value=1  ids_nominal_unit=A  vds_specify=off  vds_priority=None  vds=0 V  vds_nominal_specify=off  vds_nominal_value=1  vds_nominal_unit=V  vgs_specify=off  vgs_priority=None  vgs=0 V  vgs_nominal_specify=off  vgs_nominal_value=1  vgs_nominal_unit=V  thermal_loss_option=ee.enum.converters.thermalLossOption.tabulated2d  Von_data=[0 0.25 0.49 0.74 1.02 1.3 1.58 1.89 2.2 2.49 2.76 3.03 3.33 3.65 3.98 4.34 4.71 5.08 5.47 5.86 6.27 6.68 7.18 7.79;0 0.33 0.66 0.98 1.34 1.71 2.08 2.47 2.92 3.36 3.82 4.33 4.85 5.38 6.06 6.73 7.54 8.48 9.52 10.82 12.49 14.66 16.83 18.99] % Datasheet derived V  Tj=[25 175] % Datasheet derived degC  Iout_data=[0 4.34 8.68 13.02 17.36 21.69 26.03 30.37 34.71 39.05 43.39 47.73 52.07 56.41 60.74 65.08 69.42 73.76 78.1 82.44 86.78 91.12 95.46 99.79] % Datasheet derived A  tabulateWithVds=false % Parameter not set  Eon_data=[48.85 51.27 53.69 56.12 58.54 60.96 63.38 65.81 68.23 70.65 73.07 75.5 77.92 80.34 82.76 85.19 87.61 90.03 92.45 96.36 101.18 106.01 110.83 115.66 120.48 125.3 130.13 134.95 139.78 144.6 149.42 154.25 160.12 167.74 175.35 182.96 190.58 198.19 205.81 213.42 221.04 228.65 236.26 243.88 251.49 259.11 266.72 278.95 292.18 305.42 318.66 331.89 345.13 358.37 371.61 384.84 398.08 411.32 424.56 439.44 457.69 475.94 494.19 512.43 530.68 548.93 568.13 588.61 609.09 629.57 650.05 670.53] % Datasheet derived uJ  Eoff_data=[31.1 31.28 31.47 31.66 31.84 32.03 32.21 32.4 32.58 32.77 32.96 33.14 33.33 33.51 33.7 33.89 34.07 37.14 40.34 43.53 46.72 49.91 53.1 56.29 59.48 62.68 65.87 69.67 75.6 81.53 87.46 93.39 99.32 105.25 111.18 117.11 123.04 128.97 134.9 141.66 148.96 156.26 163.56 170.86 178.16 185.46 192.76 200.06 207.36 214.66 222.22 231.42 240.63 249.83 259.04 268.24 277.45 286.65 295.86 305.06 314.27 323.6 332.99 342.39 351.78 361.17 370.56 379.95 389.35 398.74 408.13 417.52] % Datasheet derived uJ  Eon_data_3D=[zeros(2, 5, 3)] % Parameter not set J  Eoff_data_3D=[zeros(2, 5, 3)] % Parameter not set J  Tj_loss=25 % Datasheet derived degC  Iout_data_loss=[0 1.12 2.24 3.36 4.47 5.59 6.71 7.83 8.95 10.07 11.18 12.3 13.42 14.54 15.66 16.78 17.9 19.01 20.13 21.25 22.37 23.49 24.61 25.72 26.84 27.96 29.08 30.2 31.32 32.44 33.55 34.67 35.79 36.91 38.03 39.15 40.26 41.38 42.5 43.62 44.74 45.86 46.97 48.09 49.21 50.33 51.45 52.57 53.69 54.8 55.92 57.04 58.16 59.28 60.4 61.51 62.63 63.75 64.87 65.99 67.11 68.23 69.34 70.46 71.58 72.7 73.82 74.94 76.05 77.17 78.29 79.41] % Datasheet derived A  Vds_loss=[0, 150, 300] % Parameter not set V  Eon_scalar=22.86e-3 % Parameter not set J  Eoff_scalar=17.14e-3 % Parameter not set J  Voff=400 % Datasheet derived V  Iout_scalar=600 % Parameter not set A  useCurrentFromPreviousCycle=false % Parameter not set  useVoltageFromPreviousCycle=false % Parameter not set  diodeModelType=ee.enum.converters.diodeModelType.tabulated  diodeTableType=ee.enum.diode.tableType.IfMat  diode_ReverseIVType=ee.enum.diode.diodeReverseIV.constant  diode_IfMat=[0 0.1665 0.2493 2.6035 11.0361 27.1534 51.6742 89.05;0 0.3874 0.8255 4.4328 17.0798 39.5683 67.6172 103.3819] % Datasheet derived A  diode_VfMat=[.9, 1.15, 1.25, 1.5, 1.75, 2.17, 2.6, 2.85; .58, .68, .75, 1.1, 1.38, 1.77, 2.27, 2.7] % Parameter not set V  diode_TjVec=[25 175] % Datasheet derived degC  diode_VfVec=[0 1 1.99 2.99 3.98 4.98 5.97 6.97] % Datasheet derived V  diode_IfVec=[.1, .2, .5, 1, 2, 4, 7, 10] % Parameter not set A  diode_IrMat=[1e-06, 2e-06, 5e-06, 1e-05, 2.5e-05, 5e-05, .0001; 2e-06, 5e-06, 1e-05, 4e-05, 8e-05, .0002, .0005] % Parameter not set A  diode_VrMat=[10, 100, 200, 250, 300, 325, 350; 10, 70, 160, 220, 270, 300, 320] % Parameter not set V  diode_VrVec=[10, 20, 40, 50, 70, 80, 100] % Parameter not set V  diode_IrVec=[1e-06, 2e-06, 5e-06, 1e-05, 2e-05, 5e-05, .0001] % Parameter not set A  diode_Vr=-600 % Parameter not set V  diode_Ls=150 % Parameter not set nH  diode_Erec=0.03 % Parameter not set J  diode_rec_loss_model=ee.enum.diode.reverseRecoveryModel.fixed  diode_ErecVal=0 % Parameter not set J  diode_scaleWithIandV=false  diode_ErecMat=zeros(2, 3) % Parameter not set J  diodeErecMat3D=zeros(2, 3, 2) J  diode_TjrecVec=[298.15, 398.15] % Parameter not set K  diode_IfrecVec=[.1, 1, 10] % Parameter not set A  diodeVrecVec=[0, 100] V  diode_IrecVal=10 % Parameter not set A  diode_VrecVal=10 % Parameter not set V  diode_tFilter=1 / 1000 / 100 % Parameter not set s  separateThermalPortForDiode=false % Parameter not set  thermal_network_parameterization=ee.enum.thermalNetworkTopology.external  Rth=[.03, .2] % Parameter not set K/W  Rth_Cauer=[.03, .1, .2] % Parameter not set K/W  Rth_Foster=[.08, .14, .22, .16] % Parameter not set K/W  thermal_mass_parameterization=ee.enum.thermalNetwork.timeconstant  thermal_mass=[3, 25] % Parameter not set J/K  thermal_mass_Cauer=[3, 10, 25] % Parameter not set J/K  thermal_mass_Foster=[.001, .005, .05, .5] % Parameter not set J/K  thermal_time_constant=[.1, 5] % Parameter not set s  thermal_time_constant_Cauer=[.1, 1, 5] % Parameter not set s  thermal_time_constant_Foster=[7e-05, .0007, .01, .08] % Parameter not set s  thermal_mass_initial_temperatures=[25, 25] % Parameter not set degC  thermal_mass_initial_temperatures_Cauer=[25, 25, 25] % Parameter not set degC  junction_thermal_mass=1.29 % Datasheet derived J/K  Tvec_initial_Foster=[25, 25, 25, 25] % Parameter not set degC  RthDiode=[.03, .2] % Parameter not set K/W  RthCauerDiode=[.03, .1, .2] % Parameter not set K/W  RthFosterDiode=[.03, .2] % Parameter not set K/W  thermalMassDiode=[3, 25] % Parameter not set J/K  thermalMassCauerDiode=[3, 10, 25] % Parameter not set J/K  thermalMassFosterDiode=[33, 50] % Parameter not set J/K  thermalTauDiode=[.1, 5] % Parameter not set s  thermalTauCauerDiode=[.1, 1, 5] % Parameter not set s  thermalTauFosterDiode=[1, 10] % Parameter not set s  thermalMassInitTempDiode=[25, 25] % Parameter not set degC  thermalMassInitTempCauerDiode=[25, 25, 25] % Parameter not set degC  junctionthermalMassDiode=0.1 % Parameter not set J/K  TVecInitialFosterDiode=[25, 25, 25, 25] % Parameter not set degC  no_thermal_network=0 % Parameter not set  mosfet_junction_temperature_specify=on  mosfet_junction_temperature_priority=High  mosfet_junction_temperature=simTempPri_K K  mosfet_junction_temperature_nominal_specify=off  mosfet_junction_temperature_nominal_value=1  mosfet_junction_temperature_nominal_unit=degC  diode_junction_temperature_specify=off  diode_junction_temperature_priority=None  diode_junction_temperature=simTempPri_K K  diode_junction_temperature_nominal_specify=off  diode_junction_temperature_nominal_value=1  diode_junction_temperature_nominal_unit=degC  Qj_specify=off  Qj_priority=None  Qj=0 W  Qj_nominal_specify=off  Qj_nominal_value=1  Qj_nominal_unit=W  accumulatedSwitchingLosses_specify=off  accumulatedSwitchingLosses_priority=None  accumulatedSwitchingLosses=0 J
      settings: AttributesFormatString=STMicroelectronics:SCTH35N65G2V-7
  Simulink-PS Converter{1..4} (4 alike) : nesl_utility/Simulink-PS Converter  PhysicalDomain=network_engine_domain  SubClassName=ps_input  LeftPortType=input  RightPortType=output  PseudoPeriodic=off  Frequencies=[]  NoiseDistribution=none  NoiseParameters=[]  Unit=1  AffineConversion=off  FilteringAndDerivatives=provide  SimscapeFilterOrder=1  InputFilterTimeConstant=0.001  UdotUserProvided=0
  Temperature Source{,1..3} (4 alike) : fl_lib/Thermal/Thermal Sources/Temperature Source  temperature=simTempPri_K K
  Thermal Resistor{,1..3} (4 alike) : ee_lib/Passive/Thermal/Thermal Resistor  R=1e-4 K/W  T_specify=off  T_priority=None  T=0 K  T_nominal_specify=off  T_nominal_value=1  T_nominal_unit=K  Q_specify=off  Q_priority=None  Q=0 W  Q_nominal_specify=off  Q_nominal_value=1  Q_nominal_unit=W
  P1 : PMIOPort  Side=Left
  N1 : PMIOPort  Port=2  Side=Left
  P2 : PMIOPort  Port=3  Side=Right
  N2 : PMIOPort  Port=4  Side=Right
  wires:
  G1/1 -> Simulink-PS Converter4/1
  G3/1 -> Simulink-PS Converter2/1
  G4/1 -> Simulink-PS Converter3/1
  G2/1 -> Simulink-PS Converter1/1
  connections:
  P1/RConn1 -- MOSFETB1/RConn1 -- Cds1/LConn1 -- Cds/LConn1 -- MOSFETA1/RConn1
  Cds3/LConn1 -- P2/RConn1 -- MOSFETA1/RConn2 -- Cds/RConn1 -- MOSFETA2/RConn1
  Simulink-PS Converter4/RConn1 -- MOSFETA1/LConn1
  Thermal Resistor/LConn1 -- Temperature Source/LConn1
  Thermal Resistor/RConn1 -- MOSFETA1/LConn2
  Cds2/LConn1 -- MOSFETB2/RConn1 -- N2/RConn1 -- MOSFETB1/RConn2 -- Cds1/RConn1
  Thermal Resistor1/RConn1 -- MOSFETB1/LConn2
  Simulink-PS Converter2/RConn1 -- MOSFETB1/LConn1
  Thermal Resistor1/LConn1 -- Temperature Source1/LConn1
  Thermal Resistor2/RConn1 -- MOSFETB2/LConn2
  Simulink-PS Converter3/RConn1 -- MOSFETB2/LConn1
  Thermal Resistor2/LConn1 -- Temperature Source2/LConn1
  Thermal Resistor3/RConn1 -- MOSFETA2/LConn2
  Simulink-PS Converter1/RConn1 -- MOSFETA2/LConn1
  Thermal Resistor3/LConn1 -- Temperature Source3/LConn1
  Cds2/RConn1 -- Cds3/RConn1 -- N1/RConn1 -- MOSFETA2/RConn2 -- MOSFETB2/RConn2
